simulink model "ur3_model"  (R2022a)
settings: Solver=FixedStepAuto  StartTime=0.0  StopTime=11  FixedStep=0.001  RelTol=1e-3
undefined symbols (not defined in the file): X, Y, Z
libraries: sm_lib x211, nesl_utility x27
(part 5 of 5)

== matlab function ur3_model/Inverse Jacobian1 ==
  settings: updateMethod=DISCRETE
  data: dx input; output_joint_value output; dy input; dz input; d_alpha input; d_beta input; d_gamma input; joint_value input; output_djoint_value output; det_J output
% function [dt1,dt2,dt3,dt4,dt5,dt6] = fcn(dx,dy,dz,d_alpha,d_beta,d_gamma, joint_value)
function [output_joint_value,output_djoint_value,det_J]  = fcn(dx,dy,dz,d_alpha,d_beta,d_gamma, joint_value)
% persistent theta1 theta2 theta3 theta4 theta5 theta6
% if isempty(theta1)
%     theta1 =  1e-5;
%     theta2 =  1e-5;
%     theta3 =  1e-5;
%     theta4 =  1e-5;
%     theta5 =  1e-5;
%     theta6 =  1e-5;    
% end

% constant parameters
d3= 0.15;
a2 = 0.4318;
a3 = 0.0203;
d4 = 0.4318;
d5 = 0.1;
dt =0.01;

if (length(joint_value)>1)
    t1 = joint_value(1);
    t2 = joint_value(2);
    t3 = joint_value(3);
    t4 = joint_value(4);
    t5 = joint_value(5);
    t6 = joint_value(6);
else
    t1 =  1e-5;
    t2 =  1e-5;
    t3 =  1e-5;
    t4 =  1e-5;
    t5 =  1e-5;
    t6 =  1e-5;
end

j_matrix = zeros(6,6);

j_matrix(1,1) = (2253*cos(t1))/20000 + (819*cos(t1)*cos(t5))/10000 + (4873*cos(t2)*sin(t1))/20000 - (853*sin(t1)*sin(t2)*sin(t3))/4000 + (819*cos(t2 + t3 + t4)*sin(t1)*sin(t5))/10000 - (1707*cos(t2 + t3)*sin(t1)*sin(t4))/20000 - (1707*sin(t2 + t3)*cos(t4)*sin(t1))/20000 + (853*cos(t2)*cos(t3)*sin(t1))/4000;

j_matrix(1,2) = (cos(t1)*(1707*cos(t2 + t3 + t4) - 819*cos(t2 + t3 + t4 + t5) + 4265*sin(t2 + t3) + 4873*sin(t2) + 819*cos(t2 + t3 + t4 - t5)))/20000;

j_matrix(1,3) = (cos(t1)*(1707*cos(t2 + t3 + t4) - 819*cos(t2 + t3 + t4 + t5) + 4265*sin(t2 + t3) + 819*cos(t2 + t3 + t4 - t5)))/20000;

j_matrix(1,4) = (3*cos(t1)*(546*sin(t2 + t3 + t4)*sin(t5) - 569*sin(t2 + t3)*sin(t4) + 569*cos(t2 + t3)*cos(t4)))/20000;

j_matrix(1,5) = - (819*sin(t1)*sin(t5))/10000 - (819*cos(t2 + t3 + t4)*cos(t1)*cos(t5))/10000;

j_matrix(1,6) = 0;

j_matrix(2,1) = (2253*sin(t1))/20000 - (4873*cos(t1)*cos(t2))/20000 + (819*cos(t5)*sin(t1))/10000 + (853*cos(t1)*sin(t2)*sin(t3))/4000 - (819*cos(t2 + t3 + t4)*cos(t1)*sin(t5))/10000 + (1707*cos(t2 + t3)*cos(t1)*sin(t4))/20000 + (1707*sin(t2 + t3)*cos(t1)*cos(t4))/20000 - (853*cos(t1)*cos(t2)*cos(t3))/4000;

j_matrix(2,2) = (sin(t1)*(1707*cos(t2 + t3 + t4) - 819*cos(t2 + t3 + t4 + t5) + 4265*sin(t2 + t3) + 4873*sin(t2) + 819*cos(t2 + t3 + t4 - t5)))/20000;

j_matrix(2,3) = (sin(t1)*(1707*cos(t2 + t3 + t4) - 819*cos(t2 + t3 + t4 + t5) + 4265*sin(t2 + t3) + 819*cos(t2 + t3 + t4 - t5)))/20000;

j_matrix(2,4) = (3*sin(t1)*(546*sin(t2 + t3 + t4)*sin(t5) - 569*sin(t2 + t3)*sin(t4) + 569*cos(t2 + t3)*cos(t4)))/20000;

j_matrix(2,5) = (819*cos(t1)*sin(t5))/10000 - (819*cos(t2 + t3 + t4)*cos(t5)*sin(t1))/10000;

j_matrix(2,6) = 0;


j_matrix(3,1) = 0;

j_matrix(3,2) = sin(t5)*((819*sin(t2 + t3)*sin(t4))/10000 - (819*cos(t2 + t3)*cos(t4))/10000) - (4873*cos(t2))/20000 - (853*cos(t2 + t3))/4000 + (1707*cos(t2 + t3)*sin(t4))/20000 + (1707*sin(t2 + t3)*cos(t4))/20000;

j_matrix(3,3) = (1707*sin(t2 + t3 + t4))/20000 - (853*cos(t2 + t3))/4000 - (819*cos(t2 + t3 + t4)*sin(t5))/10000;

j_matrix(3,4) = (1707*sin(t2 + t3 + t4))/20000 - (819*cos(t2 + t3 + t4)*sin(t5))/10000;

j_matrix(3,5) = -(819*sin(t2 + t3 + t4)*cos(t5))/10000;

j_matrix(3,6) = 0;


j_matrix(4,1) = 0;

j_matrix(4,2) = sin(t1);

j_matrix(4,3) = sin(t1);

j_matrix(4,4) =  sin(t1);

j_matrix(4,5) = sin(t2 + t3 + t4)*cos(t1);

j_matrix(4,6) = cos(t5)*sin(t1) - cos(t2 + t3 + t4)*cos(t1)*sin(t5);

j_matrix(5,1) = 0;

j_matrix(5,2) = -cos(t1);

j_matrix(5,3) = -cos(t1);

j_matrix(5,4) =  -cos(t1);

j_matrix(5,5) = sin(t2 + t3 + t4)*sin(t1);

j_matrix(5,6) = - cos(t1)*cos(t5) - cos(t2 + t3 + t4)*sin(t1)*sin(t5);

j_matrix(6,1) = 1;

j_matrix(6,2) = 0;

j_matrix(6,3) = 0;

j_matrix(6,4) = 0;

j_matrix(6,5) = -cos(t2 + t3 + t4);

j_matrix(6,6) = -sin(t2 + t3 + t4)*sin(t5);

d_ef = [dx dy dz d_alpha d_beta d_gamma]';

%d_joint = inv(j_matrix)*d_ef;
d_joint = j_matrix\d_ef;


dt1 = d_joint(1);
dt2 = d_joint(2);
dt3 = d_joint(3);
dt4 = d_joint(4);
dt5 = d_joint(5);
dt6 = d_joint(6);


output_joint_value =zeros(6,1);

output_joint_value(1) = dt1 + t1;
output_joint_value(2) = dt2 + t2;
output_joint_value(3) = dt3 + t3;
output_joint_value(4) = dt4 + t4;
output_joint_value(5) = dt5 + t5;
output_joint_value(6) = dt6 + t6;

output_djoint_value =zeros(6,1);

output_djoint_value(1) = dt1;
output_djoint_value(2) = dt2;
output_djoint_value(3) = dt3;
output_djoint_value(4) = dt4;
output_djoint_value(5) = dt5;
output_djoint_value(6) = dt6;

% J = j_matrix;
det_J = det(j_matrix);

== matlab function ur3_model/ur3kinematic ==
  data: x output; t1 input; y output; t2 input; t3 input; t4 input; t5 input; t6 input; z output; R output
function [x,y,z,R] = fcn(t1,t2,t3,t4,t5,t6)

% Constant params
% d3= 0.15;
% a2 = 0.4318;
% a3 = 0.0203;
% d4 = 0.4318;
% d5 = 0.1;

% end effector position
x = (4873*cos(t2)*cos((pi*((180*t1)/pi + 180))/180))/20000 - (2253*sin((pi*((180*t1)/pi + 180))/180))/20000 - (819*sin((pi*((180*t1)/pi + 180))/180)*cos(t5))/10000 - (819*sin(t5)*(cos((pi*((180*t4)/pi + 180))/180)*(cos(t2)*cos(t3)*cos((pi*((180*t1)/pi + 180))/180) - sin(t2)*sin(t3)*cos((pi*((180*t1)/pi + 180))/180)) - sin((pi*((180*t4)/pi + 180))/180)*(cos(t2)*sin(t3)*cos((pi*((180*t1)/pi + 180))/180) + cos(t3)*sin(t2)*cos((pi*((180*t1)/pi + 180))/180))))/10000 + (1707*cos((pi*((180*t4)/pi + 180))/180)*(cos(t2)*sin(t3)*cos((pi*((180*t1)/pi + 180))/180) + cos(t3)*sin(t2)*cos((pi*((180*t1)/pi + 180))/180)))/20000 + (1707*sin((pi*((180*t4)/pi + 180))/180)*(cos(t2)*cos(t3)*cos((pi*((180*t1)/pi + 180))/180) - sin(t2)*sin(t3)*cos((pi*((180*t1)/pi + 180))/180)))/20000 + (853*cos(t2)*cos(t3)*cos((pi*((180*t1)/pi + 180))/180))/4000 - (853*sin(t2)*sin(t3)*cos((pi*((180*t1)/pi + 180))/180))/4000;

 
y = (2253*cos((pi*((180*t1)/pi + 180))/180))/20000 + (1707*sin((pi*((180*t4)/pi + 180))/180)*(sin((pi*((180*t1)/pi + 180))/180)*cos(t2)*cos(t3) - sin((pi*((180*t1)/pi + 180))/180)*sin(t2)*sin(t3)))/20000 + (819*cos(t5)*cos((pi*((180*t1)/pi + 180))/180))/10000 + (4873*sin((pi*((180*t1)/pi + 180))/180)*cos(t2))/20000 + (819*sin(t5)*(sin((pi*((180*t4)/pi + 180))/180)*(sin((pi*((180*t1)/pi + 180))/180)*cos(t2)*sin(t3) + sin((pi*((180*t1)/pi + 180))/180)*cos(t3)*sin(t2)) - cos((pi*((180*t4)/pi + 180))/180)*(sin((pi*((180*t1)/pi + 180))/180)*cos(t2)*cos(t3) - sin((pi*((180*t1)/pi + 180))/180)*sin(t2)*sin(t3))))/10000 + (1707*cos((pi*((180*t4)/pi + 180))/180)*(sin((pi*((180*t1)/pi + 180))/180)*cos(t2)*sin(t3) + sin((pi*((180*t1)/pi + 180))/180)*cos(t3)*sin(t2)))/20000 + (853*sin((pi*((180*t1)/pi + 180))/180)*cos(t2)*cos(t3))/4000 - (853*sin((pi*((180*t1)/pi + 180))/180)*sin(t2)*sin(t3))/4000;

 
z =(819*sin(t5)*(sin((pi*((180*t4)/pi + 180))/180)*(cos(t2)*cos(t3) - sin(t2)*sin(t3)) + cos((pi*((180*t4)/pi + 180))/180)*(cos(t2)*sin(t3) + cos(t3)*sin(t2))))/10000 - (1707*sin((pi*((180*t4)/pi + 180))/180)*(cos(t2)*sin(t3) + cos(t3)*sin(t2)))/20000 - (853*cos(t2)*sin(t3))/4000 - (853*cos(t3)*sin(t2))/4000 - (4873*sin(t2))/20000 + (1707*cos((pi*((180*t4)/pi + 180))/180)*(cos(t2)*cos(t3) - sin(t2)*sin(t3)))/20000 + 1519/10000;

r_matrix = zeros(3,3);

r_matrix(1,1) = - cos(t6)*(sin((pi*((180*t1)/pi + 180))/180)*sin(t5) - cos(t5)*(cos((pi*((180*t4)/pi + 180))/180)*(cos(t2)*cos(t3)*cos((pi*((180*t1)/pi + 180))/180) - sin(t2)*sin(t3)*cos((pi*((180*t1)/pi + 180))/180)) - sin((pi*((180*t4)/pi + 180))/180)*(cos(t2)*sin(t3)*cos((pi*((180*t1)/pi + 180))/180) + cos(t3)*sin(t2)*cos((pi*((180*t1)/pi + 180))/180)))) - sin(t6)*(cos((pi*((180*t4)/pi + 180))/180)*(cos(t2)*sin(t3)*cos((pi*((180*t1)/pi + 180))/180) + cos(t3)*sin(t2)*cos((pi*((180*t1)/pi + 180))/180)) + sin((pi*((180*t4)/pi + 180))/180)*(cos(t2)*cos(t3)*cos((pi*((180*t1)/pi + 180))/180) - sin(t2)*sin(t3)*cos((pi*((180*t1)/pi + 180))/180)));

r_matrix(1,2) = sin(t6)*(sin((pi*((180*t1)/pi + 180))/180)*sin(t5) - cos(t5)*(cos((pi*((180*t4)/pi + 180))/180)*(cos(t2)*cos(t3)*cos((pi*((180*t1)/pi + 180))/180) - sin(t2)*sin(t3)*cos((pi*((180*t1)/pi + 180))/180)) - sin((pi*((180*t4)/pi + 180))/180)*(cos(t2)*sin(t3)*cos((pi*((180*t1)/pi + 180))/180) + cos(t3)*sin(t2)*cos((pi*((180*t1)/pi + 180))/180)))) - cos(t6)*(cos((pi*((180*t4)/pi + 180))/180)*(cos(t2)*sin(t3)*cos((pi*((180*t1)/pi + 180))/180) + cos(t3)*sin(t2)*cos((pi*((180*t1)/pi + 180))/180)) + sin((pi*((180*t4)/pi + 180))/180)*(cos(t2)*cos(t3)*cos((pi*((180*t1)/pi + 180))/180) - sin(t2)*sin(t3)*cos((pi*((180*t1)/pi + 180))/180)));

r_matrix(1,3) = - sin((pi*((180*t1)/pi + 180))/180)*cos(t5) - sin(t5)*(cos((pi*((180*t4)/pi + 180))/180)*(cos(t2)*cos(t3)*cos((pi*((180*t1)/pi + 180))/180) - sin(t2)*sin(t3)*cos((pi*((180*t1)/pi + 180))/180)) - sin((pi*((180*t4)/pi + 180))/180)*(cos(t2)*sin(t3)*cos((pi*((180*t1)/pi + 180))/180) + cos(t3)*sin(t2)*cos((pi*((180*t1)/pi + 180))/180)));

r_matrix(2,1) = cos(t6)*(sin(t5)*cos((pi*((180*t1)/pi + 180))/180) - cos(t5)*(sin((pi*((180*t4)/pi + 180))/180)*(sin((pi*((180*t1)/pi + 180))/180)*cos(t2)*sin(t3) + sin((pi*((180*t1)/pi + 180))/180)*cos(t3)*sin(t2)) - cos((pi*((180*t4)/pi + 180))/180)*(sin((pi*((180*t1)/pi + 180))/180)*cos(t2)*cos(t3) - sin((pi*((180*t1)/pi + 180))/180)*sin(t2)*sin(t3)))) - sin(t6)*(sin((pi*((180*t4)/pi + 180))/180)*(sin((pi*((180*t1)/pi + 180))/180)*cos(t2)*cos(t3) - sin((pi*((180*t1)/pi + 180))/180)*sin(t2)*sin(t3)) + cos((pi*((180*t4)/pi + 180))/180)*(sin((pi*((180*t1)/pi + 180))/180)*cos(t2)*sin(t3) + sin((pi*((180*t1)/pi + 180))/180)*cos(t3)*sin(t2)));

r_matrix(2,2) = - sin(t6)*(sin(t5)*cos((pi*((180*t1)/pi + 180))/180) - cos(t5)*(sin((pi*((180*t4)/pi + 180))/180)*(sin((pi*((180*t1)/pi + 180))/180)*cos(t2)*sin(t3) + sin((pi*((180*t1)/pi + 180))/180)*cos(t3)*sin(t2)) - cos((pi*((180*t4)/pi + 180))/180)*(sin((pi*((180*t1)/pi + 180))/180)*cos(t2)*cos(t3) - sin((pi*((180*t1)/pi + 180))/180)*sin(t2)*sin(t3)))) - cos(t6)*(sin((pi*((180*t4)/pi + 180))/180)*(sin((pi*((180*t1)/pi + 180))/180)*cos(t2)*cos(t3) - sin((pi*((180*t1)/pi + 180))/180)*sin(t2)*sin(t3)) + cos((pi*((180*t4)/pi + 180))/180)*(sin((pi*((180*t1)/pi + 180))/180)*cos(t2)*sin(t3) + sin((pi*((180*t1)/pi + 180))/180)*cos(t3)*sin(t2)));

r_matrix(2,3) = cos(t5)*cos((pi*((180*t1)/pi + 180))/180) + sin(t5)*(sin((pi*((180*t4)/pi + 180))/180)*(sin((pi*((180*t1)/pi + 180))/180)*cos(t2)*sin(t3) + sin((pi*((180*t1)/pi + 180))/180)*cos(t3)*sin(t2)) - cos((pi*((180*t4)/pi + 180))/180)*(sin((pi*((180*t1)/pi + 180))/180)*cos(t2)*cos(t3) - sin((pi*((180*t1)/pi + 180))/180)*sin(t2)*sin(t3))); 
r_matrix(3,1) = sin(t6)*(sin((pi*((180*t4)/pi + 180))/180)*(cos(t2)*sin(t3) + cos(t3)*sin(t2)) - cos((pi*((180*t4)/pi + 180))/180)*(cos(t2)*cos(t3) - sin(t2)*sin(t3))) - cos(t5)*cos(t6)*(sin((pi*((180*t4)/pi + 180))/180)*(cos(t2)*cos(t3) - sin(t2)*sin(t3)) + cos((pi*((180*t4)/pi + 180))/180)*(cos(t2)*sin(t3) + cos(t3)*sin(t2)));

r_matrix(3,2) = cos(t6)*(sin((pi*((180*t4)/pi + 180))/180)*(cos(t2)*sin(t3) + cos(t3)*sin(t2)) - cos((pi*((180*t4)/pi + 180))/180)*(cos(t2)*cos(t3) - sin(t2)*sin(t3))) + cos(t5)*sin(t6)*(sin((pi*((180*t4)/pi + 180))/180)*(cos(t2)*cos(t3) - sin(t2)*sin(t3)) + cos((pi*((180*t4)/pi + 180))/180)*(cos(t2)*sin(t3) + cos(t3)*sin(t2)));

r_matrix(3,3) = sin(t5)*(sin((pi*((180*t4)/pi + 180))/180)*(cos(t2)*cos(t3) - sin(t2)*sin(t3)) + cos((pi*((180*t4)/pi + 180))/180)*(cos(t2)*sin(t3) + cos(t3)*sin(t2)));

R = r_matrix;
